simulink model "tanque_hil_mil_2019a"  (R2019a)
settings: Solver=VariableStepAuto  StartTime=0.0  StopTime=300  FixedStep=0.001  RelTol=1e-4
undefined symbols (not defined in the file): serial
libraries: instrumentlib x3, svdutilitieslib x1
settings Model: Creator=tom  LastModifiedBy=tom
settings DebuggingCC: SignalInfNanChecking=warning  SFMachineParentedDataDiag=error

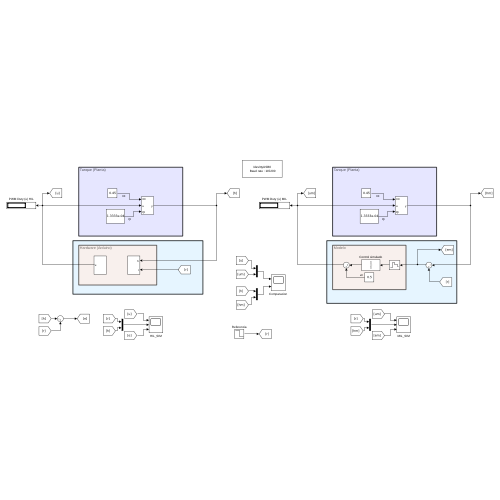
[thumbnail: Simulink's stored preview of the top-level diagram]
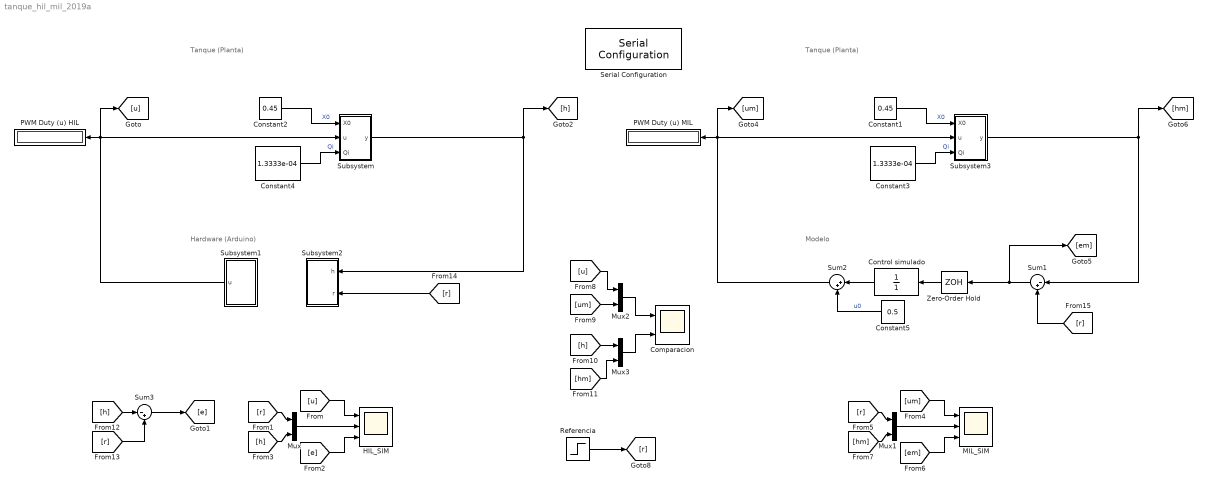
== system tanque_hil_mil_2019a ==
  note: Hardware (Arduino)
  note: Tanque (Planta)
  note: Tanque (Planta)
  note: Modelo
  Comparacion : Scope  NumInputPorts=2
  Constant1 : Constant  Value=0.45
  Constant2 : Constant  Value=0.45
  Constant3 : Constant  Value=1.3333e-04
  Constant4 : Constant  Value=1.3333e-04
  Constant5 : Constant  Value=0.5
  Control simulado : DiscreteTransferFcn  Denominator=[1]  SampleTime=1  a0EqualsOne=on  StateName=C_for
  HIL_SIM : Scope  NumInputPorts=3
  MIL_SIM : Scope  NumInputPorts=3
  Mux{,1..3} (4 alike) : Mux  Inputs=2
  PWM Duty (u) HIL : Display
      settings: Format=decimal (Stored Integer)
  PWM Duty (u) MIL : Display
      settings: Format=decimal (Stored Integer)
  Referencia : Step  Time=10  Before=0.45  After=0.4  SampleTime=0
  Serial Configuration : instrumentlib/Serial Configuration  Priority=-200000  ObjConstructor=serial('/dev/ttyUSB0');  ComPortMenu=/dev/ttyUSB0  ComPort=/dev/ttyUSB0  BaudRate=115200  DataBits=8  Parity=none  StopBits=1  ByteOrder=LittleEndian  FlowControl=none  Timeout=10
  Subsystem : Subsystem
  Subsystem1 : Subsystem
  Subsystem2 : Subsystem
  Subsystem3 : Subsystem
  Sum1 : Sum  Inputs=|-+
  Sum2 : Sum  Inputs=|++
  Sum3 : Sum  Inputs=|-+
  Zero-Order Hold : ZeroOrderHold
  wires:
  Constant2/1 -> Subsystem/1(X0)  "X0"
  Constant4/1 -> Subsystem/3(Qi)  "Qi"
  Subsystem1/1(u) -> [u], PWM Duty (u) HIL/1, Subsystem/2(u)
  Subsystem/1(y) -> Subsystem2/1(h), [h]
  [u] -> HIL_SIM/1
  Mux/1 -> HIL_SIM/2
  [e] -> HIL_SIM/3
  [r] -> Mux/1
  [h] -> Mux/2
  Subsystem3/1(y) -> [hm], Sum1/1
  [em] -> MIL_SIM/3
  [um] -> MIL_SIM/1
  Mux1/1 -> MIL_SIM/2
  [r] -> Mux1/1
  Constant1/1 -> Subsystem3/1(X0)  "X0"
  [hm] -> Mux1/2
  Constant3/1 -> Subsystem3/3(Qi)  "Qi"
  Control simulado/1 -> Sum2/1
  Constant5/1 -> Sum2/2  "u0"
  Sum2/1 -> [um], PWM Duty (u) MIL/1, Subsystem3/2(u)
  Sum1/1 -> Zero-Order Hold/1, [em]
  Zero-Order Hold/1 -> Control simulado/1
  Mux2/1 -> Comparacion/1
  [u] -> Mux2/1
  [um] -> Mux2/2
  [h] -> Mux3/1
  [hm] -> Mux3/2
  Mux3/1 -> Comparacion/2
  [h] -> Sum3/1
  Sum3/1 -> [e]
  [r] -> Sum3/2
  Referencia/1 -> [r]
  [r] -> Subsystem2/2(r)
  [r] -> Sum1/2

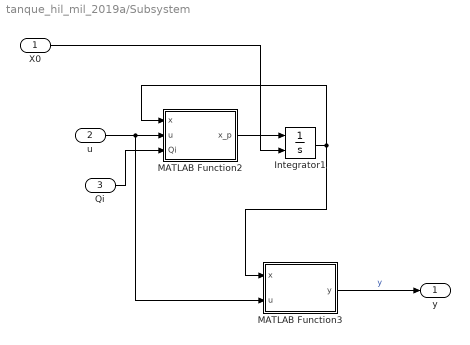
== system tanque_hil_mil_2019a/Subsystem ==
  X0 : Inport
  u : Inport  Port=2
  Qi : Inport  Port=3
  Integrator1 : Integrator  InitialConditionSource=external
  MATLAB Function2 : MATLAB Function  TreatAsAtomicUnit=on
  MATLAB Function3 : MATLAB Function  TreatAsAtomicUnit=on
  y : Outport
  wires:
  X0/1 -> Integrator1/2
  Integrator1/1 -> MATLAB Function3/1(x), MATLAB Function2/1(x)
  u/1 -> MATLAB Function3/2(u), MATLAB Function2/2(u)
  MATLAB Function2/1(x_p) -> Integrator1/1
  MATLAB Function3/1(y) -> y/1  "y"
  Qi/1 -> MATLAB Function2/3(Qi)

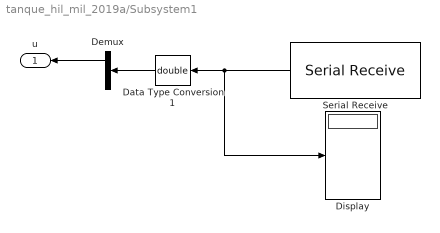
== system tanque_hil_mil_2019a/Subsystem1 ==
  Data Type Conversion1 : DataTypeConversion  OutDataTypeStr=double
  Demux : Demux  Outputs=3
  Display : Display
      settings: Format=decimal (Stored Integer)
  Serial Receive : instrumentlib/Serial Receive  ObjConstructor=serial('/dev/ttyUSB0');  ComPortMenu=/dev/ttyUSB0  ComPort=/dev/ttyUSB0  DataType=single  Header=abcd  DataSize=[3 1]  EnableBlockingMode=on  ActionDataUnavailable=Output custom value  CustomValue=-1  SampleTime=1
  u : Outport
  wires:
  Serial Receive/1 -> Display/1, Data Type Conversion1/1
  Data Type Conversion1/1 -> Demux/1
  Demux/1 -> u/1

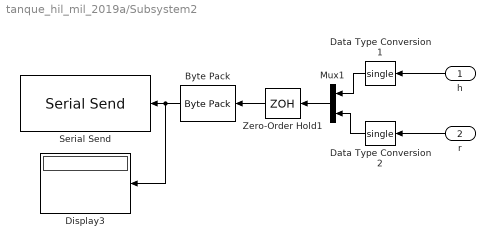
== system tanque_hil_mil_2019a/Subsystem2 ==
  h : Inport
  r : Inport  Port=2
  Byte Pack : svdutilitieslib/Byte Pack  maskPackedDataType=uint32  datatypes={'single'}  byteAlign=4  blockPlatform=arduinoert
      settings: SourceProductBaseCode=ANDROID,ARDUINO,ML_ARDUINO,ECCORTEXA,ECCORTEXR,SC_BEAGLEBONE_BLUE,EC_FREEDOM_BOARD,EC_FRDM_K64F,INTEL_BLOCKSET,MICROBIT,NUCLEO,NVIDIA,PX4AUTOPILOTS,RASPPIIO,STMICRODIS,TIC2000,XILINX_BLOCKSET
  Data Type Conversion1 : DataTypeConversion  OutDataTypeStr=single
  Data Type Conversion2 : DataTypeConversion  OutDataTypeStr=single
  Display3 : Display
      settings: Format=hex (Stored Integer)
  Mux1 : Mux  Inputs=2
  Serial Send : instrumentlib/Serial Send  ObjConstructor=serial('/dev/ttyUSB0');  ComPortMenu=/dev/ttyUSB0  ComPort=/dev/ttyUSB0  Terminator=<none>  EnableBlockingMode=on
  Zero-Order Hold1 : ZeroOrderHold
  wires:
  h/1 -> Data Type Conversion1/1
  Byte Pack/1 -> Display3/1, Serial Send/1
  Zero-Order Hold1/1 -> Byte Pack/1
  Mux1/1 -> Zero-Order Hold1/1
  Data Type Conversion2/1 -> Mux1/2
  Data Type Conversion1/1 -> Mux1/1
  r/1 -> Data Type Conversion2/1

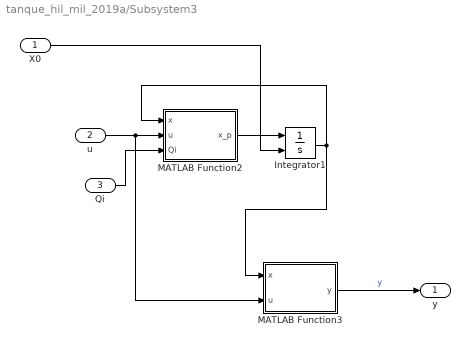
== system tanque_hil_mil_2019a/Subsystem3 ==
  X0 : Inport
  u : Inport  Port=2
  Qi : Inport  Port=3
  Integrator1 : Integrator  InitialConditionSource=external
  MATLAB Function2 : MATLAB Function  TreatAsAtomicUnit=on
  MATLAB Function3 : MATLAB Function  TreatAsAtomicUnit=on
  y : Outport
  wires:
  X0/1 -> Integrator1/2
  Integrator1/1 -> MATLAB Function3/1(x), MATLAB Function2/1(x)
  u/1 -> MATLAB Function3/2(u), MATLAB Function2/2(u)
  MATLAB Function2/1(x_p) -> Integrator1/1
  MATLAB Function3/1(y) -> y/1  "y"
  Qi/1 -> MATLAB Function2/3(Qi)

== matlab function tanque_hil_mil_2019a/Subsystem/MATLAB Function2 ==
  data: x input size=1; u input size=1; x_p output size=1; Qi input
function x_p = f(x, u, Qi)
    d = 0.01065;
    L1 = 0.1;
    L2 = 0.4;
    L = 0.9;
    g = 9.8;
    x_p = (-sqrt(abs(2*g*x))*d^2/4*u*pi + Qi)/(L1+(L2-L1)*x/L)^2;

== matlab function tanque_hil_mil_2019a/Subsystem3/MATLAB Function2 ==
  data: x input size=1; u input size=1; x_p output size=1; Qi input
function x_p = f(x, u, Qi)
    d = 0.01065;
    L1 = 0.1;
    L2 = 0.4;
    L = 0.9;
    g = 9.8;
    x_p = (-sqrt(abs(2*g*x))*d^2/4*u*pi + Qi)/(L1+(L2-L1)*x/L)^2;

== matlab function tanque_hil_mil_2019a/Subsystem3/MATLAB Function3 ==
  data: x input; u input; y output
function y = g(x, u)
    y = x;

== matlab function tanque_hil_mil_2019a/Subsystem/MATLAB Function3 ==
  data: x input; u input; y output
function y = g(x, u)
    y = x;
